simulink model "sf_battery_management"  (R2025b)
settings: Solver=FixedStepAuto  StartTime=0.0  StopTime=inf  FixedStep=0.1  RelTol=1e-3
PreLoadFcn:
  | load('battery_management_data.mat')
values from neighbouring files (symbols this model uses):
  CODEGEN_FLAG = 0    [battery_management_data.mat]
  currentFaultSim = 0    [battery_management_data.mat]
  currentSensorSim = 0    [battery_management_data.mat]
  tempFaultSim = 0    [battery_management_data.mat]
  tempSensorSim = 0    [battery_management_data.mat]
  voltageFaultSim = 0    [battery_management_data.mat]
  voltageSensorSim = 0    [battery_management_data.mat]
(part 1 of 3)
settings Model: PacingRate=10  Creator=The MathWorks, Inc.  LastModifiedBy=The MathWorks, Inc.
settings SolverCC: AlgebraicLoopSolver=TrustRegion  MaxZcPerStep=1.0
settings OptimizationCC: DefaultParameterBehavior=Inlined  EnhancedBackFolding=on  PassReuseOutputArgsAs=Individual arguments  ZeroExternalMemoryAtStartup=off  ZeroInternalMemoryAtStartup=off  OptimizeBlockOrder=speed  DifferentSizesBufferReuse=on  OptimizationCustomize=off  EfficientTunableParamExpr=on
settings DebuggingCC: ParameterTunabilityLossMsg=error  UnconnectedInputMsg=warning  UnconnectedOutputMsg=warning  UnconnectedLineMsg=warning
settings ModelReferenceCC: EnableRefExpFcnMdlSchedulingChecks=on
settings SFSimCC: MATLABDynamicMemAlloc=off
settings SFSimCC: SimCustomHeaderCode=|
  | #include "estimateSOC.h"
  | #include "batteryMonitorDriver.h"
settings SFSimCC: SimUserSources=|
  | estimateSOC.c
  | batteryMonitorDriver.c
settings RTWCC: SystemTargetFile=ert.tlc  TemplateMakefile=ert_default_tmf  GPUComputeCapability=3.5  DLArmComputeVersion=19.05  Description=Embedded Coder
settings RTWCC: CustomHeaderCode=|
  | #include "estimateSOC.h"
  | #include "batteryMonitorDriver.h"
settings RTWCC: CustomSource=|
  | estimateSOC.c
  | batteryMonitorDriver.c
settings CodeAppCC: ForceParamTrailComments=on  IgnoreCustomStorageClasses=off  OperatorAnnotations=on  SimulinkDataObjDesc=on  SFDataObjDesc=on  InsertBlockDesc=on
settings ERTTargetCC: RootIOFormat=Structure reference  ERTCustomFileTemplate=example_file_process.tlc  DynamicArrayContainerType=coder::array  TargetLangStandard=C99 (ISO)  GenerateSampleERTMain=on

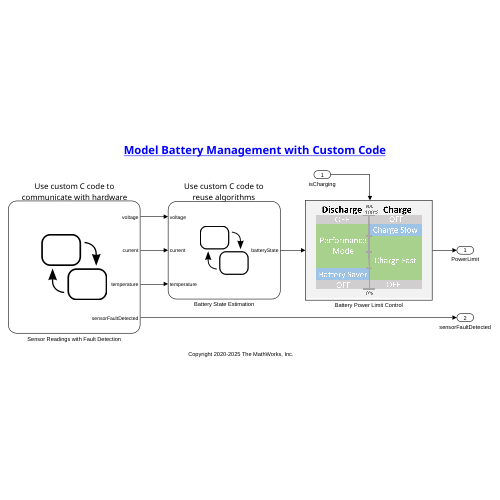
[thumbnail: Simulink's stored preview of the top-level diagram]
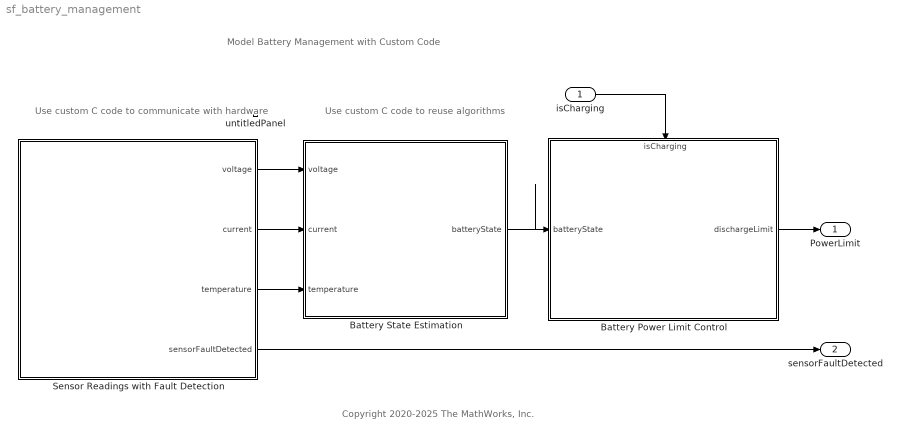
== system sf_battery_management ==
  note: Use custom C code to communicate with hardware
  note: Use custom C code to reuse algorithms
  note: Copyright 2020-2025 The MathWorks, Inc.
  note: Model Battery Management with Custom Code
  isCharging : Inport
  Battery Power Limit Control : Subsystem
      settings: PortSchema="{\"entries\":[{\"content\":{\"sides\":[{\"content\":{\"connectorIds\":[\"In1\"]},\"type\":\"ConnectorPlacement.EquallySpacedRectSide\",\"uuid\":\"80ccd787-0395-41c1-8290-ed2ee220f351\"},{\"content\":{\"connectorIds\":[\"Out1\"],\"side\":\"RIGHT\"},\"type\":\"ConnectorPlacement.EquallySpacedRectSide\",\"uuid\":\"f29d34e9-cce1-46be-963c-e76656db08b2\"},{\"content\":{\"connectorIds\":[\"In2\"],\"side\":\"TOP\"},\"type\":\"ConnectorPlacement.EquallySpacedRectSide\",\"uuid\":\"70a4eb95-761d-48a3-b772-dbe9eab67a41\"},{\"content\":{\"connectorIds\":[],\"side\":\"HIDDEN\"},\"type\":\"ConnectorPlacement.EquallySpacedRectSide\",\"uuid\":\"6c404c56-8e50-4bd8-8374-158737e1c164\"}]},\"type\":\"ConnectorPlacement.EquallySpacedConnector\",\"uuid\":\"c6965965-b0e0-4b87-babf-a4b9806b0a49\"}],\"packageUris\":[\"http://schema.mathworks.com/mf0/Connector/R2020b\"],\"version\":\"1.0\"}"
      mask Display: image('$imagefile'); % Use "Edit Image" on toolstrip to change.
  Battery State Estimation : Stateflow chart  TreatAsAtomicUnit=on
  Sensor Readings with Fault Detection : Stateflow chart  TreatAsAtomicUnit=on
  untitledPanel : Subsystem  Tag=HiddenForWebPanel  IsWebBlockPanel=on
  PowerLimit : Outport
  sensorFaultDetected : Outport  Port=2
  wires:
  Sensor Readings with Fault Detection/3(temperature) -> Battery State Estimation/3(temperature)
  Battery Power Limit Control/1(dischargeLimit) -> PowerLimit/1
  isCharging/1 -> Battery Power Limit Control/2(isCharging)
  Battery State Estimation/1(batteryState) -> Battery Power Limit Control/1(batteryState)
  Sensor Readings with Fault Detection/1(voltage) -> Battery State Estimation/1(voltage)
  Sensor Readings with Fault Detection/2(current) -> Battery State Estimation/2(current)
  Sensor Readings with Fault Detection/4(sensorFaultDetected) -> sensorFaultDetected/1

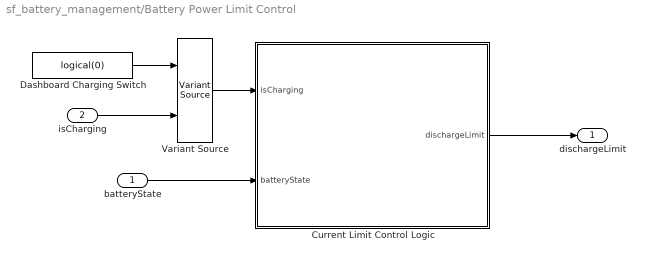
== system sf_battery_management/Battery Power Limit Control ==
  batteryState : Inport
  isCharging : Inport  Port=2
  Current Limit Control Logic : Stateflow chart  TreatAsAtomicUnit=on
  Dashboard Charging Switch : Constant  Value=logical(0)  OutDataTypeStr=boolean
  Variant Source : VariantSource  VariantControls={CODEGEN_FLAG == false, CODEGEN_FLAG == true}
  dischargeLimit : Outport
  wires:
  batteryState/1 -> Current Limit Control Logic/2(batteryState)
  Current Limit Control Logic/1(dischargeLimit) -> dischargeLimit/1
  Dashboard Charging Switch/1 -> Variant Source/1
  isCharging/1 -> Variant Source/2
  Variant Source/1 -> Current Limit Control Logic/1(isCharging)
